simulink model "NBMS_SM"  (R2026b)
settings: Solver=FixedStepDiscrete  StopTime=25  FixedStep=0.1
model workspace (MAT data in the model file):
  CAL_15_SOC_WRN_RVL_THRSH = Simulink.Parameter
  CAL_15_SOC_WRN_RVL_THRSH.Value = 15
  CAL_15_SOC_WRN_RVL_THRSH.Complexity = 'real'
  CAL_15_SOC_WRN_RVL_THRSH.Dimensions = [1 1]
  CAL_15_SOC_WRN_RVL_THRSH.DataType = 'uint8'
  CAL_15_SOC_WRN_THRSH = Simulink.Parameter
  CAL_15_SOC_WRN_THRSH.Value = 15
  CAL_15_SOC_WRN_THRSH.Complexity = 'real'
  CAL_15_SOC_WRN_THRSH.Dimensions = [1 1]
  CAL_15_SOC_WRN_THRSH.DataType = 'uint8'
  CAL_DCHRG_END_THRSH = Simulink.Parameter
  CAL_DCHRG_END_THRSH.Value = 2900
  CAL_DCHRG_END_THRSH.Complexity = 'real'
  CAL_DCHRG_END_THRSH.Dimensions = [1 1]
  CAL_DCHRG_END_THRSH.DataType = 'uint16'
  CAL_DOD = Simulink.Parameter
  CAL_DOD.Value = 100
  CAL_DOD.Complexity = 'real'
  CAL_DOD.Dimensions = [1 1]
  CAL_DOD.DataType = 'uint8'
  CAL_DOD_MAX_THRSH = Simulink.Parameter
  CAL_DOD_MAX_THRSH.Value = 99
  CAL_DOD_MAX_THRSH.Complexity = 'real'
  CAL_DOD_MAX_THRSH.Dimensions = [1 1]
  CAL_DOD_MAX_THRSH.DataType = 'uint8'
  CAL_DOD_MIN_THRSH = Simulink.Parameter
  CAL_DOD_MIN_THRSH.Value = 1
  CAL_DOD_MIN_THRSH.Complexity = 'real'
  CAL_DOD_MIN_THRSH.Dimensions = [1 1]
  CAL_DOD_MIN_THRSH.DataType = 'uint8'
  CAL_ENABLE_SOC_WARN_20 = Simulink.Parameter
  CAL_ENABLE_SOC_WARN_20.Value = 1
  CAL_ENABLE_SOC_WARN_20.Complexity = 'real'
  CAL_ENABLE_SOC_WARN_20.Dimensions = [1 1]
  CAL_ENABLE_SOC_WARN_20.DataType = 'boolean'
  CAL_GOLDEN_CHARGE = Simulink.Parameter
  CAL_GOLDEN_CHARGE.Value = 34000
  CAL_GOLDEN_CHARGE.Complexity = 'real'
  CAL_GOLDEN_CHARGE.Dimensions = [1 1]
  CAL_GOLDEN_CHARGE.DataType = 'uint16'
  CAL_GOLDEN_DC = Simulink.Parameter
  CAL_GOLDEN_DC.Value = 34000
  CAL_GOLDEN_DC.Complexity = 'real'
  CAL_GOLDEN_DC.Dimensions = [1 1]
  CAL_GOLDEN_DC.DataType = 'uint16'
  CAL_LOW_SOC_RVL_THRSH = Simulink.Parameter
  CAL_LOW_SOC_RVL_THRSH.Value = 3
  CAL_LOW_SOC_RVL_THRSH.Complexity = 'real'
  CAL_LOW_SOC_RVL_THRSH.Dimensions = [1 1]
  CAL_LOW_SOC_RVL_THRSH.DataType = 'uint8'
  CAL_LOW_SOC_THRSH = Simulink.Parameter
  CAL_LOW_SOC_THRSH.Value = 0
  CAL_LOW_SOC_THRSH.Complexity = 'real'
  CAL_LOW_SOC_THRSH.Dimensions = [1 1]
  CAL_LOW_SOC_THRSH.DataType = 'uint8'
  CAL_MOSFET_FEEDBACK = Simulink.Parameter
  CAL_MOSFET_FEEDBACK.Value = 300
  CAL_MOSFET_FEEDBACK.Complexity = 'real'
  CAL_MOSFET_FEEDBACK.Dimensions = [1 1]
  CAL_MOSFET_FEEDBACK.DataType = 'uint16'
  CAL_NOMINAL_VOLTAGE = Simulink.Parameter
  CAL_NOMINAL_VOLTAGE.Value = 101920
  CAL_NOMINAL_VOLTAGE.Complexity = 'real'
  CAL_NOMINAL_VOLTAGE.Dimensions = [1 1]
  CAL_NOMINAL_VOLTAGE.DataType = 'uint32'
  CAL_SOC_WRN_RVL_THRSH = Simulink.Parameter
  CAL_SOC_WRN_RVL_THRSH.Value = 20
  CAL_SOC_WRN_RVL_THRSH.Complexity = 'real'
  CAL_SOC_WRN_RVL_THRSH.Dimensions = [1 1]
  CAL_SOC_WRN_RVL_THRSH.DataType = 'uint8'
  CAL_SOC_WRN_THRSH = Simulink.Parameter
  CAL_SOC_WRN_THRSH.Value = 20
  CAL_SOC_WRN_THRSH.Complexity = 'real'
  CAL_SOC_WRN_THRSH.Dimensions = [1 1]
  CAL_SOC_WRN_THRSH.DataType = 'uint8'
  CAL_SOH_Enable = Simulink.Parameter
  CAL_SOH_Enable.Value = 0
  CAL_SOH_Enable.Complexity = 'real'
  CAL_SOH_Enable.Dimensions = [1 1]
  CAL_SOH_Enable.DataType = 'boolean'
  CAL_enable_SOC_warn15 = Simulink.Parameter
  CAL_enable_SOC_warn15.Value = 0
  CAL_enable_SOC_warn15.Complexity = 'real'
  CAL_enable_SOC_warn15.Dimensions = [1 1]
  CAL_enable_SOC_warn15.DataType = 'boolean'
settings Model: Creator=hp  LastModifiedBy=rathi
settings OptimizationCC: DefaultParameterBehavior=Inlined  DifferentSizesBufferReuse=on  EfficientTunableParamExpr=on  EnhancedBackFolding=on  OptimizationCustomize=off  OptimizeBlockOrder=speed  PassReuseOutputArgsAs=Individual arguments  RemoveInternalMemoryZeroInit=on  RemoveRootLevelIOMemoryZeroInit=on
settings DebuggingCC: ParameterTunabilityLossMsg=error
settings SFSimCC: MATLABDynamicMemAlloc=off
settings RTWCC: Description=Embedded Coder  GenCodeOnly=on  PackageGeneratedCodeAndArtifacts=on  SystemTargetFile=ert.tlc  TemplateMakefile=ert_default_tmf
settings CodeAppCC: ForceParamTrailComments=on  IgnoreCustomStorageClasses=off  InsertBlockDesc=on  OperatorAnnotations=on  SFDataObjDesc=on  SimulinkDataObjDesc=on
settings ERTTargetCC: DynamicArrayContainerType=coder::array  GenerateSampleERTMain=on
settings ConfigComp: DVDefectChecker=on  DVDetectOutOfBounds=on  DVHarnessSource=Signal Editor  DVModelReferenceHarness=on  DVTestSuiteOptimization=Auto

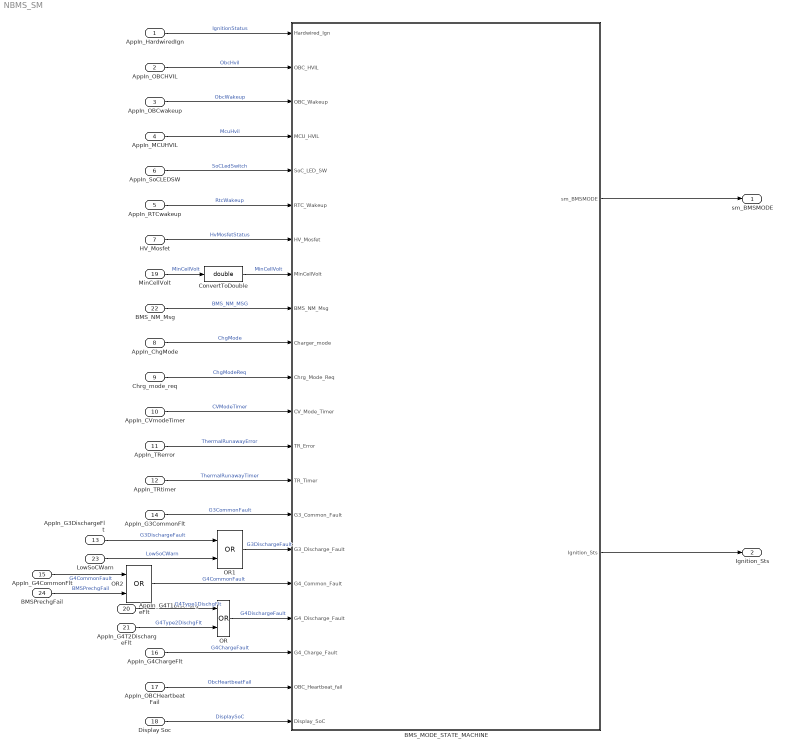
== system NBMS_SM ==
  AppIn_HardwiredIgn : Inport  OutDataTypeStr=boolean
  AppIn_OBCHVIL : Inport  Port=2  OutDataTypeStr=boolean
  AppIn_OBCwakeup : Inport  Port=3  OutDataTypeStr=Enum: OBC_E
  AppIn_MCUHVIL : Inport  Port=4  OutDataTypeStr=boolean
  AppIn_RTCwakeup : Inport  Port=5  OutDataTypeStr=boolean
  AppIn_SoCLEDSW : Inport  Port=6  OutDataTypeStr=boolean
  HV_Mosfet : Inport  Port=7  OutDataTypeStr=Enum: BMS_HVMosfet_STS_E
  AppIn_ChgMode : Inport  Port=8  OutDataTypeStr=Enum: Charger_Mode_E
  Chrg_mode_req : Inport  Port=9  OutDataTypeStr=Enum: Charger_Mode_Req_E
  AppIn_CVmodeTimer : Inport  Port=10  OutDataTypeStr=Enum: CV_Mode_Timer_E
  AppIn_TRerror : Inport  Port=11  OutDataTypeStr=boolean
  AppIn_TRtimer : Inport  Port=12  OutDataTypeStr=boolean
  AppIn_G3DischargeFlt : Inport  Port=13  OutDataTypeStr=boolean
  AppIn_G3CommonFlt : Inport  Port=14  OutDataTypeStr=boolean
  AppIn_G4CommonFlt : Inport  Port=15  OutDataTypeStr=boolean
  AppIn_G4ChargeFlt : Inport  Port=16  OutDataTypeStr=boolean
  AppIn_OBCHeartbeatFail : Inport  Port=17  OutDataTypeStr=boolean
  Display Soc : Inport  Port=18  OutDataTypeStr=uint8
  MinCellVolt : Inport  Port=19  OutDataTypeStr=fixdt(1,16,0.001,0)
  AppIn_G4T1DischargeFlt : Inport  Port=20  OutDataTypeStr=boolean
  AppIn_G4T2DischargeFlt : Inport  Port=21  OutDataTypeStr=boolean
  BMS_NM_Msg : Inport  Port=22  OutDataTypeStr=Enum: BMS_NM_Msg_E
  LowSoCWarn : Inport  Port=23
  BMSPrechgFail : Inport  Port=24
  BMS_MODE_STATE_MACHINE : Stateflow chart  TreatAsAtomicUnit=on
      settings: PortSchema="{\"entries\":[{\"content\":{\"sides\":[{\"content\":{\"connectorIds\":[\"In1\",\"In2\",\"In3\",\"In4\",\"In6\",\"In5\",\"In18\",\"In20\",\"In21\",\"In7\",\"In8\",\"In9\",\"In10\",\"In11\",\"In19\",\"In12\",\"In13\",\"In14\",\"In15\",\"In16\",\"In17\"]},\"type\":\"ConnectorPlacement.EquallySpacedRectSide\",\"uuid\":\"4784baa8-75fd-4d4e-8ae2-49fbf4d085a5\"},{\"content\":{\"connectorIds\":[\"Out1\",\"Out2\"],\"side\":\"RIGHT\"},\"type\":\"ConnectorPlacement.EquallySpacedRectSide\",\"uuid\":\"32a1afbe-c020-4b46-9ec1-8f8fc725ca88\"},{\"content\":{\"side\":\"TOP\"},\"type\":\"ConnectorPlacement.EquallySpacedRectSide\",\"uuid\":\"867b22f0-b483-4c83-be6c-4819571caf47\"}]},\"type\":\"ConnectorPlacement.EquallySpacedConnector\",\"uuid\":\"e57953f6-4ced-4f0d-9981-2e23462af30c\"}],\"packageUris\":[\"http://schema.mathworks.com/mf0/Connector/R2020b\"],\"version\":\"1.0\"}"
  ConvertToDouble : DataTypeConversion  OutDataTypeStr=double  SaturateOnIntegerOverflow=off  RndMeth=Floor
  OR : Logic  Operator=OR  AllPortsSameDT=off  OutDataTypeStr=boolean
  OR1 : Logic  Operator=OR  AllPortsSameDT=off  OutDataTypeStr=boolean
  OR2 : Logic  Operator=OR  AllPortsSameDT=off  OutDataTypeStr=boolean
  sm_BMSMODE : Outport  OutDataTypeStr=Enum: BMS_MODE_E
  Ignition_Sts : Outport  Port=2  OutDataTypeStr=boolean
  wires:
  BMS_MODE_STATE_MACHINE/1(sm_BMSMODE) -> sm_BMSMODE/1
  AppIn_ChgMode/1 -> BMS_MODE_STATE_MACHINE/7(Charger_mode)  "ChgMode"
  AppIn_TRtimer/1 -> BMS_MODE_STATE_MACHINE/11(TR_Timer)  "ThermalRunawayTimer"
  AppIn_G3DischargeFlt/1 -> OR1/1  "G3DischargeFault"
  AppIn_G4ChargeFlt/1 -> BMS_MODE_STATE_MACHINE/15(G4_Charge_Fault)  "G4ChargeFault"
  AppIn_SoCLEDSW/1 -> BMS_MODE_STATE_MACHINE/6(SoC_LED_SW)  "SoCLedSwitch"
  AppIn_G3CommonFlt/1 -> BMS_MODE_STATE_MACHINE/19(G3_Common_Fault)  "G3CommonFault"
  Chrg_mode_req/1 -> BMS_MODE_STATE_MACHINE/8(Chrg_Mode_Req)  "ChgModeReq"
  AppIn_CVmodeTimer/1 -> BMS_MODE_STATE_MACHINE/9(CV_Mode_Timer)  "CVModeTimer"
  AppIn_OBCHVIL/1 -> BMS_MODE_STATE_MACHINE/2(OBC_HVIL)  "ObcHvil"
  AppIn_OBCwakeup/1 -> BMS_MODE_STATE_MACHINE/3(OBC_Wakeup)  "ObcWakeup"
  AppIn_HardwiredIgn/1 -> BMS_MODE_STATE_MACHINE/1(Hardwired_Ign)  "IgnitionStatus"
  AppIn_MCUHVIL/1 -> BMS_MODE_STATE_MACHINE/4(MCU_HVIL)  "McuHvil"
  AppIn_TRerror/1 -> BMS_MODE_STATE_MACHINE/10(TR_Error)  "ThermalRunawayError"
  AppIn_RTCwakeup/1 -> BMS_MODE_STATE_MACHINE/5(RTC_Wakeup)  "RtcWakeup"
  OR/1 -> BMS_MODE_STATE_MACHINE/14(G4_Discharge_Fault)  "G4DischargeFault"
  AppIn_OBCHeartbeatFail/1 -> BMS_MODE_STATE_MACHINE/16(OBC_Heartbeat_fail)  "ObcHeartbeatFail"
  Display Soc/1 -> BMS_MODE_STATE_MACHINE/17(Display_SoC)  "DisplaySoC"
  HV_Mosfet/1 -> BMS_MODE_STATE_MACHINE/18(HV_Mosfet)  "HvMosfetStatus"
  MinCellVolt/1 -> ConvertToDouble/1  "MinCellVolt"
  ConvertToDouble/1 -> BMS_MODE_STATE_MACHINE/20(MinCellVolt)  "MinCellVolt"
  AppIn_G4T1DischargeFlt/1 -> OR/1  "G4Type1DischgFlt"
  AppIn_G4T2DischargeFlt/1 -> OR/2  "G4Type2DischgFlt"
  BMS_MODE_STATE_MACHINE/2(Ignition_Sts) -> Ignition_Sts/1
  BMS_NM_Msg/1 -> BMS_MODE_STATE_MACHINE/21(BMS_NM_Msg)  "BMS_NM_MSG"
  OR1/1 -> BMS_MODE_STATE_MACHINE/12(G3_Discharge_Fault)  "G3DischargeFault"
  LowSoCWarn/1 -> OR1/2  "LowSoCWarn"
  AppIn_G4CommonFlt/1 -> OR2/1  "G4CommonFault"
  BMSPrechgFail/1 -> OR2/2  "BMSPrechgFail"
  OR2/1 -> BMS_MODE_STATE_MACHINE/13(G4_Common_Fault)  "G4CommonFault"

== stateflow chart NBMS_SM/BMS_MODE_STATE_MACHINE ==
  state Sleep
    en,du,ex:
    sm_BMSMODE = BMS_MODE_E.BMS_SLEEP;
  state Standby
    en,du,ex:
    sm_BMSMODE = BMS_MODE_E.BMS_STANDBY;
  state Discharge
    en,du,ex:
    sm_BMSMODE = BMS_MODE_E.BMS_DISCHARGE;
  state Charge
    en,du,ex:
    sm_BMSMODE = BMS_MODE_E.BMS_CHARGE;
  state Fault
    en,du,ex:
    sm_BMSMODE = BMS_MODE_E.BMS_FAULT;
  (default) -> Sleep
  (junction 35) -> Sleep
  (junction 33) -> (junction 35)
  Sleep -> Standby : [Hardwired_Ign == true || hasChangedTo(SoC_LED_SW,1) || ...
      | (OBC_Heartbeat_fail == false && ...
      | hasChangedTo(OBC_Wakeup,OBC_E.Wake_Up)) || ...
      | hasChangedTo(RTC_Wakeup,1)]
      | {Ignition_Sts=true;}
  Standby -> Sleep [order 1] : [(Hardwired_Ign == false && HV_Mosfet == BMS_HVMosfet_STS_E.HV_DISCONNECTED) && ...
      | (RTC_Wakeup == false || OBC_Wakeup ~= OBC_E.Wake_Up) && after(10,sec)]
      | {Ignition_Sts=false;}
  Standby -> Discharge [order 4] : [Hardwired_Ign == true && OBC_HVIL == false && MCU_HVIL == true]
  Standby -> Charge [order 3] : [OBC_HVIL == true && OBC_Wakeup == OBC_E.Wake_Up && ...
      | OBC_Heartbeat_fail == false && Chrg_Mode_Req ~= Charger_Mode_Req_E.Charge_Complete && ...
      | Charger_mode ~= Charger_Mode_E.Error && Display_SoC <= 99 && MinCellVolt >= 2.25]
  Charge -> Standby [order 2] : [OBC_Heartbeat_fail == true || OBC_HVIL == false || ...
      | Chrg_Mode_Req == Charger_Mode_Req_E.Charge_Complete || ...
      | Charger_mode == Charger_Mode_E.Error || ...
      | CV_Mode_Timer == CV_Mode_Timer_E.Expired || BMS_NM_Msg == BMS_NM_Msg_E.SLEEP ]
  Discharge -> Standby [order 2] : [Hardwired_Ign == false || ...
      | (OBC_Wakeup == OBC_E.Wake_Up && OBC_Heartbeat_fail == false && ...
      | OBC_HVIL == true)]
  Standby -> Fault [order 2] : [G4_Common_Fault == true || G3_Common_Fault == true || ...
      | G4_Charge_Fault == true || G4_Discharge_Fault == true || ...
      | G3_Discharge_Fault == true]
  Fault -> Standby [order 4] : [G4_Common_Fault == false && G3_Common_Fault == false && ...
      | G4_Charge_Fault == false && G4_Discharge_Fault == false && ...
      | G3_Discharge_Fault == false]
  (junction 10) -> Discharge
  Discharge -> (junction 14) [order 1] : [G3_Common_Fault == true || G4_Discharge_Fault == true || ...
      | G3_Discharge_Fault == true || G4_Common_Fault == true]
  Charge -> (junction 21) [order 1] : [G3_Common_Fault == true || G4_Charge_Fault == true || ...
      | G4_Common_Fault == true]
  (junction 17) -> Charge
  (junction 21) -> Fault
  (junction 14) -> Fault
  Fault -> (junction 10) [order 3] : [OBC_HVIL == false && Hardwired_Ign == true && ...
      | (G4_Discharge_Fault == false && G3_Discharge_Fault == false && ...
      |  G3_Common_Fault == false && G4_Common_Fault == false)]
  Fault -> (junction 17) [order 2] : [(OBC_HVIL == true) && OBC_Wakeup == OBC_E.Wake_Up && ...
      | Charger_mode ~= Charger_Mode_E.Error && Chrg_Mode_Req ~= Charger_Mode_Req_E.Charge_Complete && ...
      | (G4_Charge_Fault == false && G3_Common_Fault == false && G4_Common_Fault == false)]
  Fault -> (junction 33) [order 1] : [(Hardwired_Ign == false && HV_Mosfet == BMS_HVMosfet_STS_E.HV_DISCONNECTED) && ...
      | ((TR_Error == false && after(10,sec)) || (TR_Error == true && TR_Timer == true))]
  data: Hardwired_Ign input; OBC_HVIL input; OBC_Wakeup input; MCU_HVIL input; RTC_Wakeup input; SoC_LED_SW input; Charger_mode input; Chrg_Mode_Req input; CV_Mode_Timer input; TR_Error input; TR_Timer input; G3_Discharge_Fault input; G4_Common_Fault input; G4_Discharge_Fault input; G4_Charge_Fault input; sm_BMSMODE output; OBC_Heartbeat_fail input; Display_SoC input; HV_Mosfet input; G3_Common_Fault input; MinCellVolt input; Ignition_Sts output; BMS_NM_Msg input
